simulink model "microduck_linear_state_feedback"  (R2026b)
settings: Solver=ode15s  StopTime=r.test.duration  MaxStep=r.p.cfg.sim.maxStep  RelTol=r.p.cfg.sim.relTol  AbsTol=r.p.cfg.sim.absTol
PreLoadFcn:
  | root=fileparts(get_param(bdroot,'FileName')); addpath(root,fullfile(root,'helpers')); md_expanded_cache;
PostLoadFcn:
  | md_sf_apply(bdroot);
InitFcn:
  | md_sf_apply(bdroot);
model workspace (MAT data in the model file):
  A = [0 0 0 0 0 0 0 0 0 0 0 0 ... (1296 elements, 36x36)]
  B = [0  0  0  0  0  0  0  0; 0  0  0  0  0  0  0  0; 0  0  0  0  0  0  0  0; 0  0  0  0  0  0  0  0; 0  0  0  0  0  0  0  0; 0  0  0  0  0  0  0  0; 0  0  0  0  0  0  0  0; 0  0  0  0  0  0  0  0; 0  0  0  0  0  0  0  0; 0  0  0  0  0  0  0  0; 0  0  0  0  0  0  0  0; 0  0  0  0  0  0  0  0; 0  0  0  0  0  0  0  0; 0  0  0  0  0  0  0  0; 0  0  0  0  0  0  0  0; 0  0  0  0  0  0  0  0; 0  0  0  0  0  0  0  0; 0  0  0  0  0  0  0  0; 0  0  0  0  0  0  0  0; 0  0  0  0  0  0  0  0; 0  0  0  0  0  0  0  0; 0  0  0  0  0  0  0  0; 0  0  0  0  0  0  0  0; 0  0  0  0  0  0  0  0; 0  0  0  0  0  0  0  0; 0  0  0  0  0  0  0  0; 0  0  0  0  0  0  0  0; 0  0  0  0  0  0  0  0; 18.3333333333  0  0  0  0  0  0  0; 0  18.3333333328  0  0  0  0  0  0; 0  0  18.3333333339  0  0  0  0  0; 0  0  0  18.3333333328  0  0  0  0; 0  0  0  0  18.3333333333  0  0  0; 0  0  0  0  0  18.3333333328  0  0; 0  0  0  0  0  0  18.3333333339  0; 0  0  0  0  0  0  0  18.3333333328]
  C = [0 0 0 0 0 0 0 0 0 0 0 0 ... (504 elements, 14x36)]
  E = [0  0  0  0  0  0; 0  0  0  0  0  0; 0  0  0  0  0  0; 0  0  0  0  0  0; 0  0  0  0  0  0; 0  0  0  0  0  0; 0  0  0  0  0  0; 0  0  0  0  0  0; 0  0  0  0  0  0; 0  0  0  0  0  0; 0  0  0  0  0  0; 0  0  0  0  0  0; 0  0  0  0  0  0; 0  0  0  0  0  0; 2.99982286451  -1.39842679811e-16  0.177414688657  -4.57651764544e-15  -30.0277204497  6.50739104523e-15; -1.58268629198e-16  2.89225820935  6.70083365122e-17  26.4522242149  3.51536253633e-15  -2.99721816856; 0.177414688663  8.37728579002e-17  1.49617665797  1.51751719319e-15  -1.96848927847  1.08542064426e-15; 6.08932332349e-15  -2.9843307487  6.98022045066e-16  -46.5047890403  -1.8610446411e-13  1033.95442638; -30.0277204497  3.01733642702e-15  -1.9684892784  9.66057478592e-14  670.762570803  -1.79597476519e-13; -2.99085236462e-15  26.4522273543  1.22764163289e-15  571.194337556  6.97130001697e-14  -46.7830781998; 4.28916538281e-15  -58.9426085695  -3.230112201e-15  -867.400266402  -9.48911648967e-14  29.6379320526; 93.8758569341  20.513888201  31.4835453095  429.750563248  -1381.35416373  -794.127195927; -48.639015031  -44.7564909477  -63.6327672593  -957.446876757  541.099997319  595.256445506; -27.6741686092  33.1017153167  46.5274762001  722.046276778  308.318673607  358.193155987; 4.44518421763e-15  -58.9426085695  -2.95924669915e-15  -867.400266402  -9.69858375627e-14  29.6379320526; 93.8758569341  -20.513888201  31.4835453095  -429.750563248  -1381.35416373  794.127195927; -48.639015031  44.7564909477  -63.6327672593  957.446876757  541.099997319  -595.256445506; -27.6741686092  -33.1017153167  46.5274762001  -722.046276778  308.318673607  -358.193155987; 0  0  0  0  0  0; 0  0  0  0  0  0; 0  0  0  0  0  0; 0  0  0  0  0  0; 0  0  0  0  0  0; 0  0  0  0  0  0; 0  0  0  0  0  0; 0  0  0  0  0  0]
  F_w = [0  0  0  0  0  0; 0  0  0  0  0  0; 0  0  0  0  0  0; 1.49835005027  0  0.0782612723698  0  3.51137069423  0; 2.66705636347e-18  1.56957414393  9.97031711871e-17  -2.1086255103  -9.94861602458e-17  -0.632877334553; 0.178876169343  0  1.49626291615  0  -1.98311843072  0; 0  0  0  0  0  0; 0  0  0  0  0  0; 0  0  0  0  0  0; 0  0  0  0  0  0; 0  0  0  0  0  0; 0  0  0  0  0  0; 0  0  0  0  0  0; 0  0  0  0  0  0]
  push_wrench = [1; 0; 0; 0; 0; 0]
  r.p.cfg.robot.gravity = [0; 0; -9.81]
  r.p.cfg.robot.hipHalfSpacing = 0.04
  r.p.cfg.robot.hipPitchDrop = 0.01
  r.p.cfg.robot.thighLength = 0.05
  r.p.cfg.robot.shinLength = 0.05
  r.p.cfg.robot.thighWidth = 0.025
  r.p.cfg.robot.shinWidth = 0.022
  r.p.cfg.robot.footLength = 0.054
  r.p.cfg.robot.footWidth = 0.041
  r.p.cfg.robot.footThickness = 0.012
  r.p.cfg.robot.soleDepth = 0.018
  r.p.cfg.robot.torsoDimensions = [0.09; 0.1; 0.14]
  r.p.cfg.robot.imuOffset = [0; 0; 0.05]
  r.p.cfg.robot.torsoCOM = [0; 0; 0.055]
  r.p.cfg.robot.carrierDimensions = [0.025; 0.025; 0.02]
  r.p.cfg.robot.massTorso = 0.5045154
  r.p.cfg.robot.massCarrier = 0.0287231
  r.p.cfg.robot.massThigh = 0.04315
  r.p.cfg.robot.massShin = 0.0215844
  r.p.cfg.robot.massFoot = 0.02646535
  r.p.cfg.robot.standingJointDeg = [0; -20; 40; -20; 0; -20; 40; -20]
  r.p.cfg.servo.kp = [0.55; 0.55; 0.55; 0.55; 0.55; 0.55; 0.55; 0.55]
  r.p.cfg.servo.kd = [0; 0; 0; 0; 0; 0; 0; 0]
  r.p.cfg.servo.timeConstant = [0.03; 0.03; 0.03; 0.03; 0.03; 0.03; 0.03; 0.03]
  r.p.cfg.servo.maxTorque = [0.6; 0.6; 0.6; 0.6; 0.6; 0.6; 0.6; 0.6]
  r.p.cfg.servo.jointDamping = [0.053; 0.053; 0.053; 0.053; 0.053; 0.053; 0.053; 0.053]
  r.p.cfg.servo.minCommandDeg = [-20.0535228296; -57.2957795131; 2.86478897565; -45.8366236105; -20.0535228296; -57.2957795131; 2.86478897565; -45.8366236105]
  r.p.cfg.servo.maxCommandDeg = [20.0535228296; 34.3774677078; 85.9436692696; 45.8366236105; 20.0535228296; 34.3774677078; 85.9436692696; 45.8366236105]
  r.p.cfg.contact.stiffness = 4000
  r.p.cfg.contact.damping = 12
  r.p.cfg.contact.friction = 0.6
  r.p.cfg.contact.frictionVelocity = 0.005
  r.p.cfg.sim.sampleTime = 0.02
  r.p.cfg.sim.stopTime = 3
  r.p.cfg.sim.maxStep = 0.002
  r.p.cfg.sim.relTol = 1e-06
  r.p.cfg.sim.absTol = 1e-08
  r.p.cfg.stop.enabled = 1
  r.p.cfg.stop.maxTiltDeg = 20
  r.p.cfg.stop.minHipHeight = 0.06
  r.p.cfg.measurements.includeJointVelocity = 0
  r.p.g = [0; 0; -9.81]
  r.p.nq = 14
  r.p.S = [0  0  0  0  0  0  0  0; 0  0  0  0  0  0  0  0; 0  0  0  0  0  0  0  0; 0  0  0  0  0  0  0  0; 0  0  0  0  0  0  0  0; 0  0  0  0  0  0  0  0; 1  0  0  0  0  0  0  0; 0  1  0  0  0  0  0  0; 0  0  1  0  0  0  0  0; 0  0  0  1  0  0  0  0; 0  0  0  0  1  0  0  0; 0  0  0  0  0  1  0  0; 0  0  0  0  0  0  1  0; 0  0  0  0  0  0  0  1]
  r.p.kp = [0.55; 0.55; 0.55; 0.55; 0.55; 0.55; 0.55; 0.55]
  r.p.kd = [0; 0; 0; 0; 0; 0; 0; 0]
  r.p.Ta = [0.03; 0.03; 0.03; 0.03; 0.03; 0.03; 0.03; 0.03]
  r.p.tauMax = [0.6; 0.6; 0.6; 0.6; 0.6; 0.6; 0.6; 0.6]
  r.p.bjoint = [0.053; 0.053; 0.053; 0.053; 0.053; 0.053; 0.053; 0.053]
  r.p.jointMin = [-0.35; -1; 0.05; -0.8; -0.35; -1; 0.05; -0.8]
  r.p.jointMax = [0.35; 0.6; 1.5; 0.8; 0.35; 0.6; 1.5; 0.8]
  r.p.kn = 4000
  r.p.cn = 12
  r.p.mu = 0.6
  r.p.vs = 0.005
  r.p.imuOffset = [0; 0; 0.05]
  r.p.parent = [0 1 2 3 4 1 6 7 8]
  r.p.jointIndex = [0 7 8 9 10 11 12 13 14]
  r.p.axis = [0  1  0  0  0  1  0  0  0; 0  0  1  1  1  0  1  1  1; 0  0  0  0  0  0  0  0  0]
  r.p.offset = [0  0  0  0  0  0  0  0  0; 0  0.04  0  0  0  -0.04  0  0  0; 0  0  -0.01  -0.05  -0.05  0  -0.01  -0.05  -0.05]
  r.p.mass = [0.5045154 0.0287231 0.04315 0.0215844 0.02646535 0.0287231 0.04315 0.0215844 0.02646535]
  r.p.com = [0  0  0  0  0  0  0  0  0; 0  0  0  0  0  0  0  0  0; 0.055  -0.005  -0.025  -0.025  -0.012  -0.005  -0.025  -0.025  -0.012]
  r.p.inertia = reshape([0.00124447132 0 0 0 0.001164589715 0 0 0 0.000760977395 2.45343145833e-06 0 0 0 2.45343145833e-06 0 0 0 2.99198958333e-06 1.12369791667e-05 0 0 0 1.12369791667e-05 0 0 0 4.49479166667e-06 5.3673208e-06 0 0 0 5.3673208e-06 0 0 0 1.7411416e-06 4.02493864583e-06 0 0 0 6.74866425e-06 0 0 0 1.01384344958e-05 2.45343145833e-06 0 0 0 2.45343145833e-06 0 0 0 2.99198958333e-06 1.12369791667e-05 0 0 0 1.12369791667e-05 0 0 0 4.49479166667e-06 5.3673208e-06 0 0 0 5.3673208e-06 0 0 0 1.7411416e-06 4.02493864583e-06 0 0 0 6.74866425e-06 0 0 0 1.01384344958e-05], [3 3 9])
  r.p.footBodies = [5 9]
  r.p.corners = [-0.027  -0.027  0.027  0.027; -0.0205  0.0205  -0.0205  0.0205; -0.018  -0.018  -0.018  -0.018]
  r.p.qnom = [0; 0; 0.121741068879; 0; 0; 0; 0; -0.349065850399; 0.698131700798; -0.349065850399; 0; -0.349065850399; 0.698131700798; -0.349065850399]
  r.p.trimResidual = 3.34843264227e-13
  r.p.trimNormal = [0.86015562883; 0.86015562883; 0.96538996892; 0.96538996892; 0.86015562883; 0.86015562883; 0.96538996892; 0.96538996892]
  r.p.xeq = [0; 0; 0.121741054404; 0; 0.00048719603821; 6.28632250353e-17; 0; -0.349065850399; 0.698131700798; -0.349065850399; 0; -0.349065850399; 0.698131700798; -0.349065850399; 0; 0; 0; 0; 0; 0; 0; 0; 0; 0; 0; 0; 0; 0; 5.52116353176e-16; 7.90529085794e-05; -0.0506100270862; 0.00565215320243; 5.52116353176e-16; 7.90529085794e-05; -0.0506100270862; 0.00565215320243]
  r.p.ueq = [1.00384791487e-15; -0.348922117838; 0.606113469732; -0.338789208213; 1.00384791487e-15; -0.348922117838; 0.606113469732; -0.338789208213]
  r.lin.A = [0 0 0 0 0 0 0 0 0 0 0 0 ... (1296 elements, 36x36)]
  r.lin.B = [0  0  0  0  0  0  0  0; 0  0  0  0  0  0  0  0; 0  0  0  0  0  0  0  0; 0  0  0  0  0  0  0  0; 0  0  0  0  0  0  0  0; 0  0  0  0  0  0  0  0; 0  0  0  0  0  0  0  0; 0  0  0  0  0  0  0  0; 0  0  0  0  0  0  0  0; 0  0  0  0  0  0  0  0; 0  0  0  0  0  0  0  0; 0  0  0  0  0  0  0  0; 0  0  0  0  0  0  0  0; 0  0  0  0  0  0  0  0; 0  0  0  0  0  0  0  0; 0  0  0  0  0  0  0  0; 0  0  0  0  0  0  0  0; 0  0  0  0  0  0  0  0; 0  0  0  0  0  0  0  0; 0  0  0  0  0  0  0  0; 0  0  0  0  0  0  0  0; 0  0  0  0  0  0  0  0; 0  0  0  0  0  0  0  0; 0  0  0  0  0  0  0  0; 0  0  0  0  0  0  0  0; 0  0  0  0  0  0  0  0; 0  0  0  0  0  0  0  0; 0  0  0  0  0  0  0  0; 18.3333333333  0  0  0  0  0  0  0; 0  18.3333333328  0  0  0  0  0  0; 0  0  18.3333333339  0  0  0  0  0; 0  0  0  18.3333333328  0  0  0  0; 0  0  0  0  18.3333333333  0  0  0; 0  0  0  0  0  18.3333333328  0  0; 0  0  0  0  0  0  18.3333333339  0; 0  0  0  0  0  0  0  18.3333333328]
  r.lin.C = [0  0  0  0  0  0  0  0  0  0  0  0  0  0  0  0  0  -0.000487196018936  0  1  0  0  0  0  0  0  0  0  0  0  0  0  0  0  0  0; 0  0  0  0  0  0  0  0  0  0  0  0  0  0  0  0  0  6.28632175747e-17  1  5.73971850987e-36  0  0  0  0  0  0  0  0  0  0  0  0  0  0  0  0; 0  0  0  0  0  0  0  0  0  0  0  0  0  0  0  0  0  0.99999988132  -6.28632250353e-17  0  0  0  0  0  0  0  0  0  0  0  0  0  0  0  0  0; 0  0  9265.46457746  0  130.165054704  -6.84001466578e-08  -2.07256087292e-09  69.3951978499  144.565706863  64.1932730965  -2.10595429984e-09  69.3951978499  144.565706863  64.1932730965  74.0137947271  0  27.7963937321  6.20163642662e-11  -8.63881750136  -1.78676518026e-10  2.86229373536e-10  -5.26342586956  -0.830679547445  0.178354369236  2.57172755314e-10  -5.26342586956  -0.830679547439  0.178354369236  0  24.7927989485  -21.5530077617  -12.2808996456  0  24.7927989485  -21.5530077617  -12.2808996456; 0  0  -7.82627372827e-11  -1.15367357622e-10  1.01085418767e-08  272.89136386  112.119374165  10.1316970194  18.6847145316  9.9177480342  112.119374165  -10.1316970296  -18.6847145316  -9.9177480442  8.21255251386e-14  515.113047543  -3.2086916701e-11  0.947725865768  -3.57478340115e-11  63.6596220389  32.5958842775  -0.557372026813  -0.482069576678  0.0855967928727  32.5958842776  0.55737202677  0.482069576771  -0.0855967928114  -15.5718784225  -0.992982191643  3.13034753722  -2.99186872359  -15.5718784225  0.992982191643  -3.13034753722  2.99186872359; 0  0  -13045.3812466  0  -291.511055468  1.00364161426e-07  4.4408920985e-09  -145.399577004  -260.915887701  -143.957256833  4.4408920985e-09  -145.399577003  -260.915887701  -143.957256832  -165.916252803  0  -39.1361437391  8.881784197e-10  19.3664195969  0  8.881784197e-10  7.18267224187  7.99488262881  -1.40613470379  0  7.18267224276  7.99488262881  -1.40613470467  0  31.5292775177  -63.6564564429  46.5139879342  0  31.5292775177  -63.6564564429  46.5139879342]
  r.lin.D = [0  0  0  0  0  0  0  0; 0  0  0  0  0  0  0  0; 0  0  0  0  0  0  0  0; 0  0  0  0  0  0  0  0; 0  0  0  0  0  0  0  0; 0  0  0  0  0  0  0  0]
  r.lin.C_with_joint_angles = [0 0 0 0 0 0 0 0 0 0 0 0 ... (504 elements, 14x36)]
  r.lin.D_with_joint_angles = [0  0  0  0  0  0  0  0; 0  0  0  0  0  0  0  0; 0  0  0  0  0  0  0  0; 0  0  0  0  0  0  0  0; 0  0  0  0  0  0  0  0; 0  0  0  0  0  0  0  0; 0  0  0  0  0  0  0  0; 0  0  0  0  0  0  0  0; 0  0  0  0  0  0  0  0; 0  0  0  0  0  0  0  0; 0  0  0  0  0  0  0  0; 0  0  0  0  0  0  0  0; 0  0  0  0  0  0  0  0; 0  0  0  0  0  0  0  0]
  r.lin.C_measurements = [0 0 0 0 0 0 0 0 0 0 0 0 ... (504 elements, 14x36)]
  r.lin.D_measurements = [0  0  0  0  0  0  0  0; 0  0  0  0  0  0  0  0; 0  0  0  0  0  0  0  0; 0  0  0  0  0  0  0  0; 0  0  0  0  0  0  0  0; 0  0  0  0  0  0  0  0; 0  0  0  0  0  0  0  0; 0  0  0  0  0  0  0  0; 0  0  0  0  0  0  0  0; 0  0  0  0  0  0  0  0; 0  0  0  0  0  0  0  0; 0  0  0  0  0  0  0  0; 0  0  0  0  0  0  0  0; 0  0  0  0  0  0  0  0]
  r.lin.xeq = [0; 0; 0.121741054404; 0; 0.00048719603821; 6.28632250353e-17; 0; -0.349065850399; 0.698131700798; -0.349065850399; 0; -0.349065850399; 0.698131700798; -0.349065850399; 0; 0; 0; 0; 0; 0; 0; 0; 0; 0; 0; 0; 0; 0; 5.52116353176e-16; 7.90529085794e-05; -0.0506100270862; 0.00565215320243; 5.52116353176e-16; 7.90529085794e-05; -0.0506100270862; 0.00565215320243]
  r.lin.ueq = [1.00384791487e-15; -0.348922117838; 0.606113469732; -0.338789208213; 1.00384791487e-15; -0.348922117838; 0.606113469732; -0.338789208213]
  r.lin.yeq = [0; 0; 0; -0.00477939294573; 2.9613909167e-15; 9.80999883575]
  r.lin.yeq_measurements = [0; 0; 0; -0.00477939294573; 2.9613909167e-15; 9.80999883575; 0; -0.349065850399; 0.698131700798; -0.349065850399; 0; -0.349065850399; 0.698131700798; -0.349065850399]
  r.lin.stateScale = [0.01; 0.01; 0.01; 0.1; 0.1; 0.1; 0.1; 0.1; 0.1; 0.1; 0.1; 0.1; 0.1; 0.1; 0.1; 0.1; 0.1; 1; 1; 1; 1; 1; 1; 1; 1; 1; 1; 1; 0.1; 0.1; 0.1; 0.1; 0.1; 0.1; 0.1; 0.1]
  r.lin.controlSampleTime = 0.02
  r.aux.E = [0  0  0  0  0  0; 0  0  0  0  0  0; 0  0  0  0  0  0; 0  0  0  0  0  0; 0  0  0  0  0  0; 0  0  0  0  0  0; 0  0  0  0  0  0; 0  0  0  0  0  0; 0  0  0  0  0  0; 0  0  0  0  0  0; 0  0  0  0  0  0; 0  0  0  0  0  0; 0  0  0  0  0  0; 0  0  0  0  0  0; 2.99982286451  -1.39842679811e-16  0.177414688657  -4.57651764544e-15  -30.0277204497  6.50739104523e-15; -1.58268629198e-16  2.89225820935  6.70083365122e-17  26.4522242149  3.51536253633e-15  -2.99721816856; 0.177414688663  8.37728579002e-17  1.49617665797  1.51751719319e-15  -1.96848927847  1.08542064426e-15; 6.08932332349e-15  -2.9843307487  6.98022045066e-16  -46.5047890403  -1.8610446411e-13  1033.95442638; -30.0277204497  3.01733642702e-15  -1.9684892784  9.66057478592e-14  670.762570803  -1.79597476519e-13; -2.99085236462e-15  26.4522273543  1.22764163289e-15  571.194337556  6.97130001697e-14  -46.7830781998; 4.28916538281e-15  -58.9426085695  -3.230112201e-15  -867.400266402  -9.48911648967e-14  29.6379320526; 93.8758569341  20.513888201  31.4835453095  429.750563248  -1381.35416373  -794.127195927; -48.639015031  -44.7564909477  -63.6327672593  -957.446876757  541.099997319  595.256445506; -27.6741686092  33.1017153167  46.5274762001  722.046276778  308.318673607  358.193155987; 4.44518421763e-15  -58.9426085695  -2.95924669915e-15  -867.400266402  -9.69858375627e-14  29.6379320526; 93.8758569341  -20.513888201  31.4835453095  -429.750563248  -1381.35416373  794.127195927; -48.639015031  44.7564909477  -63.6327672593  957.446876757  541.099997319  -595.256445506; -27.6741686092  -33.1017153167  46.5274762001  -722.046276778  308.318673607  -358.193155987; 0  0  0  0  0  0; 0  0  0  0  0  0; 0  0  0  0  0  0; 0  0  0  0  0  0; 0  0  0  0  0  0; 0  0  0  0  0  0; 0  0  0  0  0  0; 0  0  0  0  0  0]
  r.aux.Fw = [0  0  0  0  0  0; 0  0  0  0  0  0; 0  0  0  0  0  0; 1.49835005027  0  0.0782612723698  0  3.51137069423  0; 2.66705636347e-18  1.56957414393  9.97031711871e-17  -2.1086255103  -9.94861602458e-17  -0.632877334553; 0.178876169343  0  1.49626291615  0  -1.98311843072  0; 0  0  0  0  0  0; 0  0  0  0  0  0; 0  0  0  0  0  0; 0  0  0  0  0  0; 0  0  0  0  0  0; 0  0  0  0  0  0; 0  0  0  0  0  0; 0  0  0  0  0  0]
  r.feedback.K = [8.70410247674e-16 -0.000482616394029 -0.000818546928294 -0.00100799621853 -3.20893583014e-15 -0.000482616394022 -0.000818546928299 -0.00100799621853 3.94214592664e-14 -0.0216180096191 -0.0366654667942 -0.0451515369514 ... (264 elements, 8x33)]
  r.feedback.poles = [-0.173706973501+0.0790896944051i; -0.173706973501-0.0790896944051i; -0.014115987547+0.0894236107172i; -0.014115987547-0.0894236107172i; 0.672250176228+0.561912229918i; 0.672250176228-0.561912229918i; -0.0822703613827+0.0594677475137i; -0.0822703613827-0.0594677475137i; 0.0992828819218+0i; 0.891684694096+0i; 0.886920436717+0i; 0.735487634412+0.114439990771i; 0.735487634412-0.114439990771i; 0.717373000186+0.112026826557i; 0.717373000186-0.112026826557i; 0.976285709758+0i; 0.980198673307+0i; 0.721801481118+0.118511971968i; 0.721801481118-0.118511971968i; 0.482156928981+0i; 0.480371127775+0i; 0.492850316995+0i; 0.515715029329+0i; 0.514305187301+0i; 2.94698823164e-09+0i; -5.41379190099e-16+0i; 1.47117542566e-16+0i; 1.11020150478e-17+9.9609496806e-17i; 1.11020150478e-17-9.9609496806e-17i; -2.28360718307e-17+3.66102795761e-17i; -2.28360718307e-17-3.66102795761e-17i; 2.99664398283e-17+2.17653008708e-17i; 2.99664398283e-17-2.17653008708e-17i]
  r.feedback.requestedPoles = [-0.173706973501+0.0790896944051i; -0.173706973501-0.0790896944051i; -0.014115987547+0.0894236107172i; -0.014115987547-0.0894236107172i; 0.672250176228+0.561912229918i; 0.672250176228-0.561912229918i; -0.0822703613827+0.0594677475137i; -0.0822703613827-0.0594677475137i; 0.0992828819218+0i; 0.891684694096+0i; 0.735487634412+0.114439990771i; 0.735487634412-0.114439990771i; 0.717373000186+0.112026826557i; 0.717373000186-0.112026826557i; 0.721801481118+0.118511971968i; 0.721801481118-0.118511971968i; 0.482156928981+0i; 0.480371127775+0i; 0.492850316995+0i; 0.515715029329+0i; 0.514305187301+0i; 2.9469884e-09+0i; 5.84077967475e-15+0i; -2.65521112042e-15+2.05477564382e-15i; -2.65521112042e-15-2.05477564382e-15i; 3.09349036794e-15+0i; 9.13638941562e-16+0i; -4.87155219894e-16+0i; 1.66967134563e-16+2.25567004766e-16i; 1.66967134563e-16-2.25567004766e-16i; 0.886920436717+0i; 0.976285709758+0i; 0.980198673307+0i]
  r.feedback.assignedSlowPoles = [0.886920436717; 0.976285709758; 0.980198673307]
  r.feedback.retainedFastPoleCount = 30
  r.feedback.poleMatchError = 1.58095758707e-13
  r.feedback.placementPrecision = 15
  r.feedback.radius = 0.980198673307
  r.feedback.reference = [0; 0]
  r.feedback.maxCorrectionRad = 0.13962634016
  r.feedback.sampleTime = 0.02
  r.observer.Ad = [-0.226035158295 0.0607901151539 1.20046417563e-11 -1.4732593899e-11 -0.156351729745 0.138229107162 0.0857639497085 -1.47317675914e-11 -0.156351729733 0.138229107138 0.0857639497232 1.19581922834 ... (1089 elements, 33x33)]
  r.observer.Bd = [-1.57872286761e-12 -2.75043555489e-12 -0.0544924598499 0.0922096305921 -0.0255771207666 0.0488604655049 -0.0163542439887 0.087766164084 0.0255771207875 -0.0488604655276 0.016354243994 1.82708257098e-11 ... (264 elements, 33x8)]
  r.observer.C = [0 0 0 9.44491801984 -7.97785293402e-14 -13.2980440841 0 0 0 0 0 0 ... (462 elements, 14x33)]
  r.observer.D = [0  0  0  0  0  0  0  0; 0  0  0  0  0  0  0  0; 0  0  0  0  0  0  0  0; 0  0  0  0  0  0  0  0; 0  0  0  0  0  0  0  0; 0  0  0  0  0  0  0  0; 0  0  0  0  0  0  0  0; 0  0  0  0  0  0  0  0; 0  0  0  0  0  0  0  0; 0  0  0  0  0  0  0  0; 0  0  0  0  0  0  0  0; 0  0  0  0  0  0  0  0; 0  0  0  0  0  0  0  0; 0  0  0  0  0  0  0  0]
  r.observer.L = [-7.01418682646e-12 8.04628712517e-11 0.0643927661333 0.24278751739 0.0372639622641 -0.0756135571544 0.0275453071133 0.242787517394 -0.0372639605356 0.07561355728 -0.0275453090267 5.98286207219e-10 ... (462 elements, 33x14)]
  r.observer.errorMatrix = [-0.251020245761 0.799832731146 2.38563787379e-09 7.04126391556e-09 2.62313977309 0.267993545053 -3.41200716347 7.0849640839e-09 2.62313976989 0.267993551207 -3.41200716574 3.40012488569 ... (1089 elements, 33x33)]
  r.observer.poles = [-0.173706973501+0.0790896944051i; -0.173706973501-0.0790896944051i; -0.014115987547+0.0894236107172i; -0.014115987547-0.0894236107172i; -0.0822703613827+0.0594677475137i; -0.0822703613827-0.0594677475137i; 0.0992828819218+0i; 0.717373000186+0.112026826557i; 0.717373000186-0.112026826557i; 0.721801481118+0.118511971968i; 0.721801481118-0.118511971968i; 0.670320046036+0i; 0.482156928981+0i; 0.582748252374+0i; 0.59452054797+0i; 0.631283645507+0i; 0.657046819815+0i; 0.644036421083+0i; 0.618783391806+0i; 0.606530659713+0i; 0.480371127775+0i; 0.492850316995+0i; 0.514305187301+0i; 0.515715029329+0i; 2.94698765516e-09+0i; 1.91663560711e-14+0i; -6.86720396472e-15+0i; -3.48279432533e-16+9.37889198838e-16i; -3.48279432533e-16-9.37889198838e-16i; 7.85859192971e-16+3.70757158126e-16i; 7.85859192971e-16-3.70757158126e-16i; -2.4574281643e-16+0i; 2.80192628595e-16+0i]
  r.observer.continuousA = [0 0 0 0 0 0 0 0 0 0 0 2088.98331426 ... (1089 elements, 33x33)]
  r.observer.continuousB = [0  0  0  0  0  0  0  0; 0  0  0  0  0  0  0  0; 0  0  0  0  0  0  0  0; 0  0  0  0  0  0  0  0; 0  0  0  0  0  0  0  0; 0  0  0  0  0  0  0  0; 0  0  0  0  0  0  0  0; 0  0  0  0  0  0  0  0; 0  0  0  0  0  0  0  0; 0  0  0  0  0  0  0  0; 0  0  0  0  0  0  0  0; 0  0  0  0  0  0  0  0; 0  0  0  0  0  0  0  0; 0  0  0  0  0  0  0  0; 0  0  0  0  0  0  0  0; 0  0  0  0  0  0  0  0; 0  0  0  0  0  0  0  0; 0  0  0  0  0  0  0  0; 0  0  0  0  0  0  0  0; 0  0  0  0  0  0  0  0; 0  0  0  0  0  0  0  0; 0  0  0  0  0  0  0  0; 0  0  0  0  0  0  0  0; 0  0  0  0  0  0  0  0; 0  0  0  0  0  0  0  0; 183.333333333  0  0  0  0  0  0  0; 0  183.333333328  0  0  0  0  0  0; 0  0  183.333333339  0  0  0  0  0; 0  0  0  183.333333328  0  0  0  0; 0  0  0  0  183.333333333  0  0  0; 0  0  0  0  0  183.333333328  0  0; 0  0  0  0  0  0  183.333333339  0; 0  0  0  0  0  0  0  183.333333328]
  r.observer.y0 = [0; 0; 0; -0.00477939294573; 2.9613909167e-15; 9.80999883575; 0; -0.349065850399; 0.698131700798; -0.349065850399; 0; -0.349065850399; 0.698131700798; -0.349065850399]
  r.observer.yScale = [1; 1; 1; 9.81; 9.81; 9.81; 0.1; 0.1; 0.1; 0.1; 0.1; 0.1; 0.1; 0.1]
  r.observer.keep = [3 5 6 7 8 9 10 11 12 13 14 15 16 17 18 19 20 21 22 23 24 25 26 27 28 29 30 31 32 33 34 35 36]
  r.observer.S = [0.01 0 0 0 0 0 0 0 0 0 0 0 ... (1089 elements, 33x33)]
  r.observer.settings.initialAngleErrorDeg = [0.5; 1]
  r.observer.settings.slowModeCutoffRate = 15
  r.observer.settings.firstDecayRate = 20
  r.observer.settings.decayRateSpacing = 1
  r.observer.settings.initialEstimateDelta = [0; 0; 0; 0; 0.0174532925199; 0.00872664625997; 0; 0; 0; 0; 0; 0; 0; 0; 0; 0; 0; 0; 0; 0; 0; 0; 0; 0; 0; 0; 0; 0; 0; 0; 0; 0; 0; 0; 0; 0]
  r.observer.sampleTime = 0.02
  r.observer.requestedSlowPoles = [0.670320046036 0.657046819815 0.644036421083 0.631283645507 0.618783391806 0.606530659713 0.59452054797 0.582748252374]
  r.observer.retainedFastPoleCount = 25
  r.observer.placementPrecision = 14
  r.test.duration = 3
  r.test.pushForce = [1; 0; 0]
  r.test.pushMoment = [0; 0; 0]
  r.test.pushCentre = 0.2
  r.test.pushWidth = 0.02
  r.test.pushEnabled = 1
  r.test.pushPointBody = [0; 0; 0]
  r.H = [0  0  1  0  0  0  0  0  0  0  0  0  0  0  0  0  0  0  0  0  0  0  0  0  0  0  0  0  0  0  0  0  0; 0  1  0  0  0  0  0  0  0  0  0  0  0  0  0  0  0  0  0  0  0  0  0  0  0  0  0  0  0  0  0  0  0]
  r.sharedConfiguration.test.duration = 3
  r.sharedConfiguration.test.pushForce = [1; 0; 0]
  r.sharedConfiguration.test.pushMoment = [0; 0; 0]
  r.sharedConfiguration.test.pushCentre = 0.2
  r.sharedConfiguration.test.pushWidth = 0.02
  r.sharedConfiguration.sampleTime = 0.02
  r.sharedConfiguration.observer.initialAngleErrorDeg = [0.5; 1]
  r.sharedConfiguration.observer.slowModeCutoffRate = 15
  r.sharedConfiguration.observer.firstDecayRate = 20
  r.sharedConfiguration.observer.decayRateSpacing = 1
  r.sharedConfiguration.robot.gravity = [0; 0; -9.81]
  r.sharedConfiguration.robot.hipHalfSpacing = 0.04
  r.sharedConfiguration.robot.hipPitchDrop = 0.01
  r.sharedConfiguration.robot.thighLength = 0.05
  r.sharedConfiguration.robot.shinLength = 0.05
  r.sharedConfiguration.robot.thighWidth = 0.025
  r.sharedConfiguration.robot.shinWidth = 0.022
  r.sharedConfiguration.robot.footLength = 0.054
  r.sharedConfiguration.robot.footWidth = 0.041
  r.sharedConfiguration.robot.footThickness = 0.012
  r.sharedConfiguration.robot.soleDepth = 0.018
  r.sharedConfiguration.robot.torsoDimensions = [0.09; 0.1; 0.14]
  r.sharedConfiguration.robot.imuOffset = [0; 0; 0.05]
  r.sharedConfiguration.robot.torsoCOM = [0; 0; 0.055]
  r.sharedConfiguration.robot.carrierDimensions = [0.025; 0.025; 0.02]
  r.sharedConfiguration.robot.massTorso = 0.5045154
  r.sharedConfiguration.robot.massCarrier = 0.0287231
  r.sharedConfiguration.robot.massThigh = 0.04315
  r.sharedConfiguration.robot.massShin = 0.0215844
  r.sharedConfiguration.robot.massFoot = 0.02646535
  r.sharedConfiguration.robot.standingJointDeg = [0; -20; 40; -20; 0; -20; 40; -20]
  r.sharedConfiguration.servo.kp = [0.55; 0.55; 0.55; 0.55; 0.55; 0.55; 0.55; 0.55]
  r.sharedConfiguration.servo.kd = [0; 0; 0; 0; 0; 0; 0; 0]
  r.sharedConfiguration.servo.timeConstant = [0.03; 0.03; 0.03; 0.03; 0.03; 0.03; 0.03; 0.03]
  r.sharedConfiguration.servo.maxTorque = [0.6; 0.6; 0.6; 0.6; 0.6; 0.6; 0.6; 0.6]
  r.sharedConfiguration.servo.jointDamping = [0.053; 0.053; 0.053; 0.053; 0.053; 0.053; 0.053; 0.053]
  r.sharedConfiguration.servo.minCommandDeg = [-20.0535228296; -57.2957795131; 2.86478897565; -45.8366236105; -20.0535228296; -57.2957795131; 2.86478897565; -45.8366236105]
  r.sharedConfiguration.servo.maxCommandDeg = [20.0535228296; 34.3774677078; 85.9436692696; 45.8366236105; 20.0535228296; 34.3774677078; 85.9436692696; 45.8366236105]
  r.sharedConfiguration.contact.stiffness = 4000
  r.sharedConfiguration.contact.damping = 12
  r.sharedConfiguration.contact.friction = 0.6
  r.sharedConfiguration.contact.frictionVelocity = 0.005
  r.sharedConfiguration.feedback.assignedDecayRates = [6; 1; 1.2]
  r.sharedConfiguration.feedback.slowModeCutoffRate = 2.5
  r.sharedConfiguration.feedback.poleMatchTolerance = 1e-06
  r.sharedConfiguration.feedback.maxCorrectionDeg = 8
  r.sharedConfiguration.solver.maxStep = 0.002
  r.sharedConfiguration.solver.relTol = 1e-06
  r.sharedConfiguration.solver.absTol = 1e-08
  r.sharedConfiguration.validity.maxTiltDeg = 20
  r.sharedConfiguration.validity.minHipHeight = 0.06
  r.sharedVersion = 1
  r.mode = 'linear'
  u_eq = [1.00384791487e-15; -0.348922117838; 0.606113469732; -0.338789208213; 1.00384791487e-15; -0.348922117838; 0.606113469732; -0.338789208213]
  x_eq = [0; 0; 0.121741054404; 0; 0.00048719603821; 6.28632250353e-17; 0; -0.349065850399; 0.698131700798; -0.349065850399; 0; -0.349065850399; 0.698131700798; -0.349065850399; 0; 0; 0; 0; 0; 0; 0; 0; 0; 0; 0; 0; 0; 0; 5.52116353176e-16; 7.90529085794e-05; -0.0506100270862; 0.00565215320243; 5.52116353176e-16; 7.90529085794e-05; -0.0506100270862; 0.00565215320243]
  y_eq = [0; 0; 0; -0.00477939294573; 2.9613909167e-15; 9.80999883575; 0; -0.349065850399; 0.698131700798; -0.349065850399; 0; -0.349065850399; 0.698131700798; -0.349065850399]
settings Model: Creator=parve  LastModifiedBy=parve

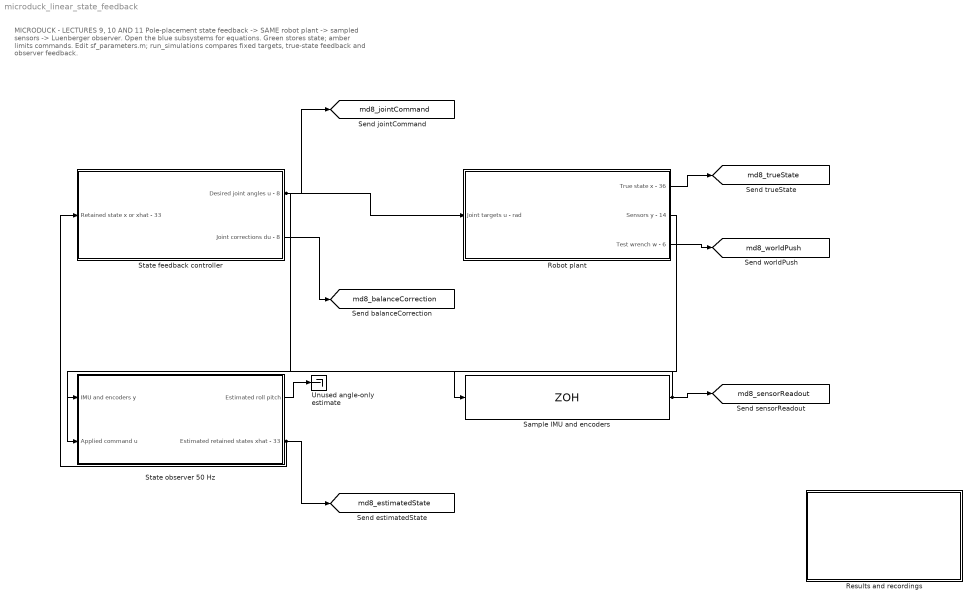
== system microduck_linear_state_feedback ==
  note: MICRODUCK - LECTURES 9, 10 AND 11
      | Pole-placement state feedback -> SAME robot plant -> sampled sensors -> Luenberger observer.
      | Open the blue subsystems for equations. Green stores state; amber limits commands.
      | Edit sf_parameters.m; run_simulations compares fixed targets, true-state feedback and observer feedback.
  Results and recordings : Subsystem  Description=|
      | RESULTS AND RECORDINGS
      | 
      | Purpose: record signals for plotting and comparison. These blocks do not control the robot.
      | trueState: actual motion; estimatedState: observer output; jointCommand: applied targets.
      | sensorReadout, worldPush and balanceCorrection complete the experiment records.
      mask help:
      | RESULTS AND RECORDINGS
      |
      | Purpose: record signals for plotting and comparison. These blocks do not control the robot.
      | trueState: actual motion; estimatedState: observer output; jointCommand: applied targets.
      | sensorReadout, worldPush and balanceCorrection complete the experiment records.
      settings: OpenFcn=open_system(gcb,'force');
      mask Display: disp('Results and recordings');
  Robot plant : Subsystem  Description=|
      | LINEAR PLANT - SMALL CHANGES ABOUT STANDING
      | 
      | Purpose: approximate the robot near its standing equilibrium.
      | State derivative = A * state deviation + B * command deviation + E * push.
      | The integrator stores state deviations; add standing offsets to reconstruct physical outputs.
      mask help:
      | LINEAR PLANT - SMALL CHANGES ABOUT STANDING
      |
      | Purpose: approximate the robot near its standing equilibrium.
      | State derivative = A * state deviation + B * command deviation + E * push.
      | The integrator stores state deviations; add standing offsets to reconstruct physical outputs.
      settings: OpenFcn=open_system(gcb,'force');
      mask Display: disp('Robot plant');
  Sample IMU and encoders : ZeroOrderHold  Description=|  SampleTime=r.observer.sampleTime
      | Sample IMU and encoders
      | 
      | WHAT THIS BLOCK DOES
      | Samples the sensor signal every 0.02 s and holds that measurement between samples, representing the 50 Hz readout clock.
      | 
      | FOLDER CONTEXT
      | MICRODUCK BALANCE - START HERE
      | 
      | Follow the loop: state-feedback controller -> robot plant -> sampled sensors -> observer -> PID.
      | Open a folder for its purpose, signal meanings and equations. Green blocks store state; amber blocks limit signals.
      | The controller and observer update at 50 Hz. Results are recorded separately on the right.
  State feedback controller : Subsystem  Description=Lecture 9 pole-placement feedback. Normalize standing state deviations, apply -K, limit offsets, and add standing joint targets.
      settings: OpenFcn=open_system(gcb,'force');
      mask Display: disp('State feedback controller\nLecture 9: pole placement')
  State observer 50 Hz : Subsystem  Description=|
      | Lecture 10 Luenberger observer, sampled as in Lecture 11.
      | zhat[k+1]=Ad zhat[k]+Bd du[k]+L(yn[k]-Cn zhat[k]).
      | The same applied joint target is sent to both plant and observer.
      settings: OpenFcn=open_system(gcb,'force');
      mask Display: disp('State observer\nLuenberger pole placement')
  Unused angle-only estimate : Terminator
  tag scope: md8_balanceCorrection=global, md8_estimatedState=global, md8_jointCommand=global, md8_sensorReadout=global, md8_trueState=global, md8_worldPush=global
  wires:
  State feedback controller/1(Desired joint angles u - 8) -> Robot plant/1(Joint targets u - rad), State observer 50 Hz/2(Applied command u), [md8_jointCommand]
  State feedback controller/2(Joint corrections du - 8) -> [md8_balanceCorrection]
  Robot plant/1(True state x - 36) -> [md8_trueState]
  Robot plant/2(Sensors y - 14) -> Sample IMU and encoders/1
  Robot plant/3(Test wrench w - 6) -> [md8_worldPush]
  Sample IMU and encoders/1 -> State observer 50 Hz/1(IMU and encoders y), [md8_sensorReadout]
  State observer 50 Hz/2(Estimated retained states xhat - 33) -> State feedback controller/1(Retained state x or xhat - 33), [md8_estimatedState]
  State observer 50 Hz/1(Estimated roll pitch) -> Unused angle-only estimate/1

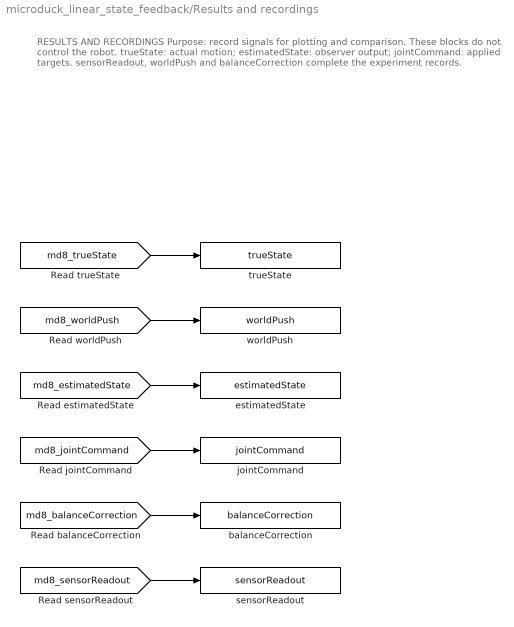
== system microduck_linear_state_feedback/Results and recordings ==
  note: RESULTS AND RECORDINGS
      |
      | Purpose: record signals for plotting and comparison. These blocks do not control the robot.
      | trueState: actual motion; estimatedState: observer output; jointCommand: applied targets.
      | sensorReadout, worldPush and balanceCorrection complete the experiment records.
  balanceCorrection : ToWorkspace  VariableName=balanceCorrection  SaveFormat=Timeseries  SampleTime=-1
      settings: Description=|
      | balanceCorrection
      | 
      | WHAT THIS BLOCK DOES
      | Records the input as a MATLAB timeseries for plots and validation. It does not feed a control action back to the robot.
      | 
      | FOLDER CONTEXT
      | RESULTS AND RECORDINGS
      | 
      | Purpose: record signals for plotting and comparison. These blocks do not control the robot.
      | trueState: actual motion; estimatedState: observer output; jointCommand: applied targets.
      | sensorReadout, worldPush and balanceCorrection complete the experiment records.
  estimatedState : ToWorkspace  VariableName=estimatedState  SaveFormat=Timeseries  SampleTime=-1
      settings: Description=|
      | estimatedState
      | 
      | WHAT THIS BLOCK DOES
      | Records the input as a MATLAB timeseries for plots and validation. It does not feed a control action back to the robot.
      | 
      | FOLDER CONTEXT
      | RESULTS AND RECORDINGS
      | 
      | Purpose: record signals for plotting and comparison. These blocks do not control the robot.
      | trueState: actual motion; estimatedState: observer output; jointCommand: applied targets.
      | sensorReadout, worldPush and balanceCorrection complete the experiment records.
  jointCommand : ToWorkspace  VariableName=jointCommand  SaveFormat=Timeseries  SampleTime=-1
      settings: Description=|
      | jointCommand
      | 
      | WHAT THIS BLOCK DOES
      | Records the input as a MATLAB timeseries for plots and validation. It does not feed a control action back to the robot.
      | 
      | FOLDER CONTEXT
      | RESULTS AND RECORDINGS
      | 
      | Purpose: record signals for plotting and comparison. These blocks do not control the robot.
      | trueState: actual motion; estimatedState: observer output; jointCommand: applied targets.
      | sensorReadout, worldPush and balanceCorrection complete the experiment records.
  sensorReadout : ToWorkspace  VariableName=sensorReadout  SaveFormat=Timeseries  SampleTime=-1
      settings: Description=|
      | sensorReadout
      | 
      | WHAT THIS BLOCK DOES
      | Records the input as a MATLAB timeseries for plots and validation. It does not feed a control action back to the robot.
      | 
      | FOLDER CONTEXT
      | RESULTS AND RECORDINGS
      | 
      | Purpose: record signals for plotting and comparison. These blocks do not control the robot.
      | trueState: actual motion; estimatedState: observer output; jointCommand: applied targets.
      | sensorReadout, worldPush and balanceCorrection complete the experiment records.
  trueState : ToWorkspace  VariableName=trueState  SaveFormat=Timeseries  SampleTime=-1
      settings: Description=|
      | trueState
      | 
      | WHAT THIS BLOCK DOES
      | Records the input as a MATLAB timeseries for plots and validation. It does not feed a control action back to the robot.
      | 
      | FOLDER CONTEXT
      | RESULTS AND RECORDINGS
      | 
      | Purpose: record signals for plotting and comparison. These blocks do not control the robot.
      | trueState: actual motion; estimatedState: observer output; jointCommand: applied targets.
      | sensorReadout, worldPush and balanceCorrection complete the experiment records.
  worldPush : ToWorkspace  VariableName=worldPush  SaveFormat=Timeseries  SampleTime=-1
      settings: Description=|
      | worldPush
      | 
      | WHAT THIS BLOCK DOES
      | Records the input as a MATLAB timeseries for plots and validation. It does not feed a control action back to the robot.
      | 
      | FOLDER CONTEXT
      | RESULTS AND RECORDINGS
      | 
      | Purpose: record signals for plotting and comparison. These blocks do not control the robot.
      | trueState: actual motion; estimatedState: observer output; jointCommand: applied targets.
      | sensorReadout, worldPush and balanceCorrection complete the experiment records.
  wires:
  [md8_balanceCorrection] -> balanceCorrection/1
  [md8_estimatedState] -> estimatedState/1
  [md8_jointCommand] -> jointCommand/1
  [md8_sensorReadout] -> sensorReadout/1
  [md8_trueState] -> trueState/1
  [md8_worldPush] -> worldPush/1

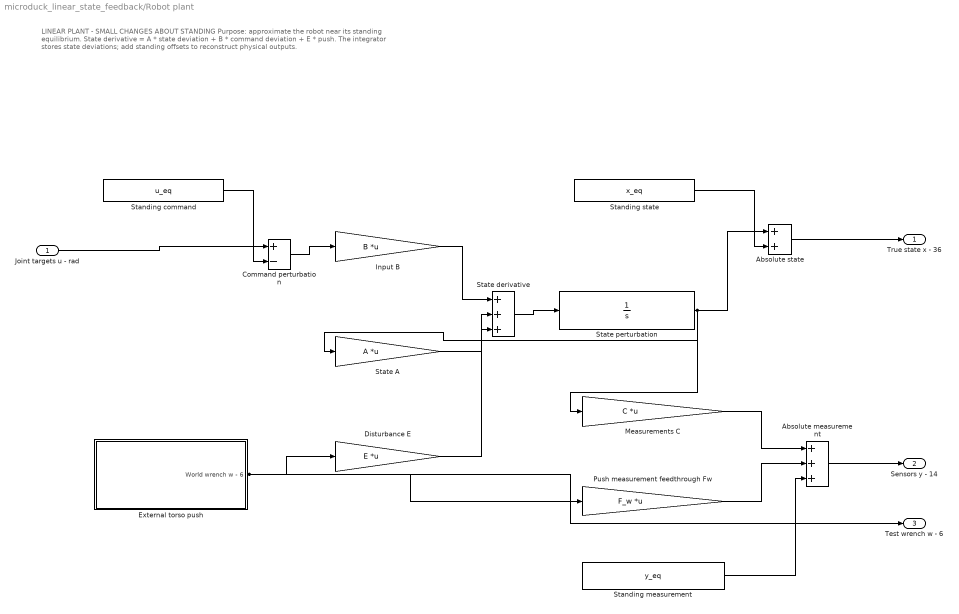
== system microduck_linear_state_feedback/Robot plant ==
  note: LINEAR PLANT - SMALL CHANGES ABOUT STANDING
      |
      | Purpose: approximate the robot near its standing equilibrium.
      | State derivative = A * state deviation + B * command deviation + E * push.
      | The integrator stores state deviations; add standing offsets to reconstruct physical outputs.
  Joint targets u - rad : Inport  Description=|
      | Joint targets u - rad
      | 
      | WHAT THIS BLOCK DOES
      | Receives this named signal from the parent folder. Check the name for its meaning and units.
      | 
      | FOLDER CONTEXT
      | LINEAR PLANT - SMALL CHANGES ABOUT STANDING
      | 
      | Purpose: approximate the robot near its standing equilibrium.
      | State derivative = A * state deviation + B * command deviation + E * push.
      | The integrator stores state deviations; add standing offsets to reconstruct physical outputs.
  Absolute measurement : Sum  Description=|  Inputs=+++
      | Absolute measurement
      | 
      | WHAT THIS BLOCK DOES
      | Combines its inputs using the plus/minus signs shown on the icon. Signs: +++.
      | 
      | FOLDER CONTEXT
      | LINEAR PLANT - SMALL CHANGES ABOUT STANDING
      | 
      | Purpose: approximate the robot near its standing equilibrium.
      | State derivative = A * state deviation + B * command deviation + E * push.
      | The integrator stores state deviations; add standing offsets to reconstruct physical outputs.
  Absolute state : Sum  Description=|
      | Absolute state
      | 
      | WHAT THIS BLOCK DOES
      | Combines its inputs using the plus/minus signs shown on the icon. Signs: ++.
      | 
      | FOLDER CONTEXT
      | LINEAR PLANT - SMALL CHANGES ABOUT STANDING
      | 
      | Purpose: approximate the robot near its standing equilibrium.
      | State derivative = A * state deviation + B * command deviation + E * push.
      | The integrator stores state deviations; add standing offsets to reconstruct physical outputs.
  Command perturbation : Sum  Description=|  Inputs=+-
      | Command perturbation
      | 
      | WHAT THIS BLOCK DOES
      | Combines its inputs using the plus/minus signs shown on the icon. Signs: +-.
      | 
      | FOLDER CONTEXT
      | LINEAR PLANT - SMALL CHANGES ABOUT STANDING
      | 
      | Purpose: approximate the robot near its standing equilibrium.
      | State derivative = A * state deviation + B * command deviation + E * push.
      | The integrator stores state deviations; add standing offsets to reconstruct physical outputs.
  Disturbance E : Gain  Description=|  Gain=E  Multiplication=Matrix(K*u)
      | SHARED PARAMETER: E = r.aux.E
      | Edit sf_parameters.m; per-model edits are refreshed on Run.
      | 
      | WHAT THIS BLOCK DOES
      | Disturbance E
      | 
      | PARAMETER
      | E = r.aux.E
      | 
      | The short symbol is stored in this model workspace. Its numeric value is unchanged from the validated model.
  External torso push : Subsystem  Description=|
      | EXTERNAL TORSO PUSH
      | 
      | Purpose: supply the repeatable disturbance used in this experiment.
      | A Gaussian 0.1 N forward push peaks at 0.2 s, with width 0.02 s.
      | It acts at the torso origin; the observer is not told this disturbance.
      mask help:
      | EXTERNAL TORSO PUSH
      |
      | Purpose: supply the repeatable disturbance used in this experiment.
      | A Gaussian 0.1 N forward push peaks at 0.2 s, with width 0.02 s.
      | It acts at the torso origin; the observer is not told this disturbance.
      settings: OpenFcn=open_system(gcb,'force');
      mask Display: disp('External torso push');
  Input B : Gain  Description=|  Gain=B  Multiplication=Matrix(K*u)
      | SHARED PARAMETER: B = r.lin.B
      | Edit sf_parameters.m; per-model edits are refreshed on Run.
      | 
      | WHAT THIS BLOCK DOES
      | Input B
      | 
      | PARAMETER
      | B = r.lin.B
      | 
      | The short symbol is stored in this model workspace. Its numeric value is unchanged from the validated model.
  Measurements C : Gain  Description=|  Gain=C  Multiplication=Matrix(K*u)
      | SHARED PARAMETER: C = r.lin.C_with_joint_angles
      | Edit sf_parameters.m; per-model edits are refreshed on Run.
      | 
      | WHAT THIS BLOCK DOES
      | Measurements C
      | 
      | PARAMETER
      | C = r.lin.C_with_joint_angles
      | 
      | The short symbol is stored in this model workspace. Its numeric value is unchanged from the validated model.
  Push measurement feedthrough Fw : Gain  Description=|  Gain=F_w  Multiplication=Matrix(K*u)
      | SHARED PARAMETER: F_w = r.aux.Fw
      | Edit sf_parameters.m; per-model edits are refreshed on Run.
      | 
      | WHAT THIS BLOCK DOES
      | Push measurement feedthrough Fw
      | 
      | PARAMETER
      | F_w = r.aux.Fw
      | 
      | The short symbol is stored in this model workspace. Its numeric value is unchanged from the validated model.
  Standing command : Constant  Description=|  Value=u_eq
      | SHARED PARAMETER: u_eq = r.p.ueq
      | Edit sf_parameters.m; per-model edits are refreshed on Run.
      | 
      | WHAT THIS BLOCK DOES
      | Standing command
      | 
      | PARAMETER
      | u_eq = r.p.ueq
      | 
      | The short symbol is stored in this model workspace. Its numeric value is unchanged from the validated model.
  Standing measurement : Constant  Description=|  Value=y_eq
      | SHARED PARAMETER: y_eq = r.observer.y0
      | Edit sf_parameters.m; per-model edits are refreshed on Run.
      | 
      | WHAT THIS BLOCK DOES
      | Standing measurement
      | 
      | PARAMETER
      | y_eq = r.observer.y0
      | 
      | The short symbol is stored in this model workspace. Its numeric value is unchanged from the validated model.
  Standing state : Constant  Description=|  Value=x_eq
      | SHARED PARAMETER: x_eq = r.p.xeq
      | Edit sf_parameters.m; per-model edits are refreshed on Run.
      | 
      | WHAT THIS BLOCK DOES
      | Standing state
      | 
      | PARAMETER
      | x_eq = r.p.xeq
      | 
      | The short symbol is stored in this model workspace. Its numeric value is unchanged from the validated model.
  State A : Gain  Description=|  Gain=A  Multiplication=Matrix(K*u)
      | SHARED PARAMETER: A = r.lin.A
      | Edit sf_parameters.m; per-model edits are refreshed on Run.
      | 
      | WHAT THIS BLOCK DOES
      | State A
      | 
      | PARAMETER
      | A = r.lin.A
      | 
      | The short symbol is stored in this model workspace. Its numeric value is unchanged from the validated model.
  State derivative : Sum  Description=|  Inputs=+++
      | State derivative
      | 
      | WHAT THIS BLOCK DOES
      | Combines its inputs using the plus/minus signs shown on the icon. Signs: +++.
      | 
      | FOLDER CONTEXT
      | LINEAR PLANT - SMALL CHANGES ABOUT STANDING
      | 
      | Purpose: approximate the robot near its standing equilibrium.
      | State derivative = A * state deviation + B * command deviation + E * push.
      | The integrator stores state deviations; add standing offsets to reconstruct physical outputs.
  State perturbation : Integrator  Description=|  InitialCondition=zeros(36,1)
      | State perturbation
      | 
      | WHAT THIS BLOCK DOES
      | Continuous state memory: integrates the input over time. Starts at InitialCondition = zeros(36,1).
      | 
      | FOLDER CONTEXT
      | LINEAR PLANT - SMALL CHANGES ABOUT STANDING
      | 
      | Purpose: approximate the robot near its standing equilibrium.
      | State derivative = A * state deviation + B * command deviation + E * push.
      | The integrator stores state deviations; add standing offsets to reconstruct physical outputs.
  True state x - 36 : Outport  Description=|
      | True state x - 36
      | 
      | WHAT THIS BLOCK DOES
      | Carries this named result out of the folder. The port number defines the interface order.
      | 
      | FOLDER CONTEXT
      | LINEAR PLANT - SMALL CHANGES ABOUT STANDING
      | 
      | Purpose: approximate the robot near its standing equilibrium.
      | State derivative = A * state deviation + B * command deviation + E * push.
      | The integrator stores state deviations; add standing offsets to reconstruct physical outputs.
  Sensors y - 14 : Outport  Description=|  Port=2
      | Sensors y - 14
      | 
      | WHAT THIS BLOCK DOES
      | Carries this named result out of the folder. The port number defines the interface order.
      | 
      | FOLDER CONTEXT
      | LINEAR PLANT - SMALL CHANGES ABOUT STANDING
      | 
      | Purpose: approximate the robot near its standing equilibrium.
      | State derivative = A * state deviation + B * command deviation + E * push.
      | The integrator stores state deviations; add standing offsets to reconstruct physical outputs.
  Test wrench w - 6 : Outport  Description=|  Port=3
      | Test wrench w - 6
      | 
      | WHAT THIS BLOCK DOES
      | Carries this named result out of the folder. The port number defines the interface order.
      | 
      | FOLDER CONTEXT
      | LINEAR PLANT - SMALL CHANGES ABOUT STANDING
      | 
      | Purpose: approximate the robot near its standing equilibrium.
      | State derivative = A * state deviation + B * command deviation + E * push.
      | The integrator stores state deviations; add standing offsets to reconstruct physical outputs.
  wires:
  Measurements C/1 -> Absolute measurement/1
  Push measurement feedthrough Fw/1 -> Absolute measurement/2
  Standing measurement/1 -> Absolute measurement/3
  State perturbation/1 -> Absolute state/1, Measurements C/1, State A/1
  Standing state/1 -> Absolute state/2
  Joint targets u - rad/1 -> Command perturbation/1
  Standing command/1 -> Command perturbation/2
  External torso push/1(World wrench w - 6) -> Disturbance E/1, Push measurement feedthrough Fw/1, Test wrench w - 6/1
  Command perturbation/1 -> Input B/1
  Input B/1 -> State derivative/1
  State A/1 -> State derivative/2
  Disturbance E/1 -> State derivative/3
  State derivative/1 -> State perturbation/1
  Absolute state/1 -> True state x - 36/1
  Absolute measurement/1 -> Sensors y - 14/1

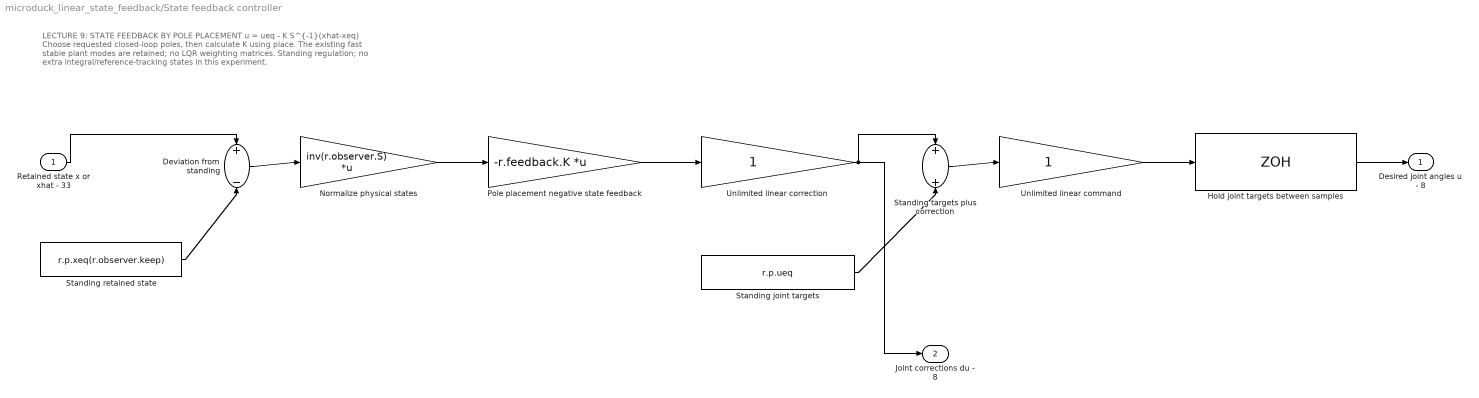
== system microduck_linear_state_feedback/State feedback controller ==
  note: LECTURE 9: STATE FEEDBACK BY POLE PLACEMENT
      | u = ueq - K S^{-1}(xhat-xeq)
      | Choose requested closed-loop poles, then calculate K using place.
      | The existing fast stable plant modes are retained; no LQR weighting matrices.
      | Standing regulation; no extra integral/reference-tracking states in this experiment.
  Retained state x or xhat - 33 : Inport
  Deviation from standing : Sum  Inputs=+-
  Hold joint targets between samples : ZeroOrderHold  Description=Digital controller period Ts. Its input is sampled at the same period as the observer and true-state baseline.  SampleTime=r.observer.sampleTime
  Normalize physical states : Gain  Description=z = S^(-1)*(x-xeq). Scaling makes metres, radians, rates and torques comparable in the LQR cost.  Gain=inv(r.observer.S)  Multiplication=Matrix(K*u)
  Pole placement negative state feedback : Gain  Description=du = -K*z. K is calculated using pole placement in equivalent state coordinates; no LQR cost or weights are used.  Gain=-r.feedback.K  Multiplication=Matrix(K*u)
  Standing joint targets : Constant  Value=r.p.ueq
  Standing retained state : Constant  Value=r.p.xeq(r.observer.keep)
  Standing targets plus correction : Sum
  Unlimited linear command : Gain
  Unlimited linear correction : Gain  Description=The local linear baseline bypasses nonlinear limits, matching the earlier linear plant architecture.
  Desired joint angles u - 8 : Outport
  Joint corrections du - 8 : Outport  Port=2
  wires:
  Retained state x or xhat - 33/1 -> Deviation from standing/1
  Standing retained state/1 -> Deviation from standing/2
  Deviation from standing/1 -> Normalize physical states/1
  Normalize physical states/1 -> Pole placement negative state feedback/1
  Pole placement negative state feedback/1 -> Unlimited linear correction/1
  Unlimited linear correction/1 -> Standing targets plus correction/1, Joint corrections du - 8/1
  Standing joint targets/1 -> Standing targets plus correction/2
  Standing targets plus correction/1 -> Unlimited linear command/1
  Unlimited linear command/1 -> Hold joint targets between samples/1
  Hold joint targets between samples/1 -> Desired joint angles u - 8/1

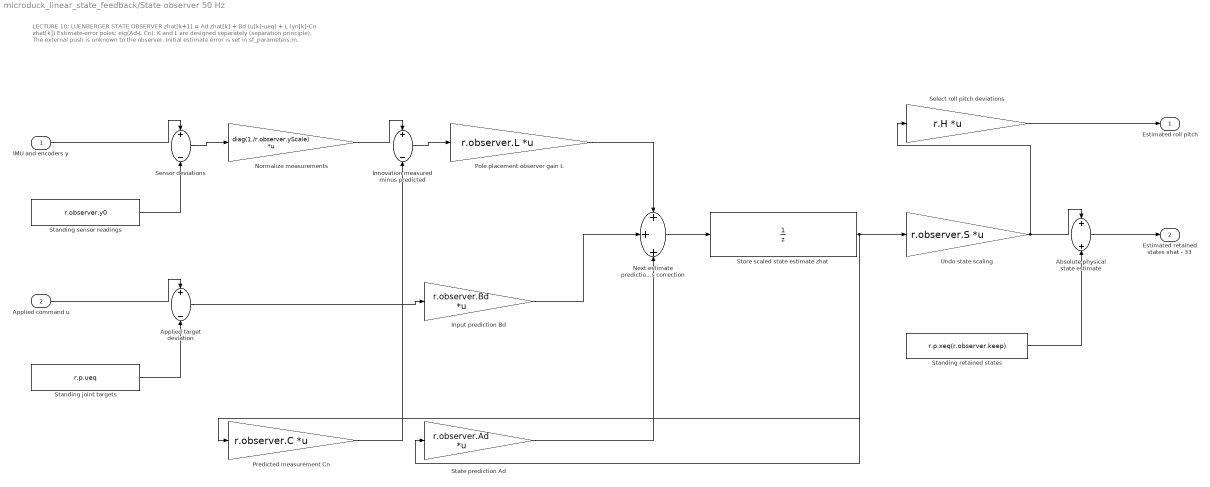
== system microduck_linear_state_feedback/State observer 50 Hz ==
  note: LECTURE 10: LUENBERGER STATE OBSERVER
      | zhat[k+1] = Ad zhat[k] + Bd (u[k]-ueq) + L (yn[k]-Cn zhat[k])
      | Estimate-error poles: eig(Ad-L Cn). K and L are designed separately (separation principle).
      | The external push is unknown to the observer. Initial estimate error is set in sf_parameters.m.
  IMU and encoders y : Inport
  Applied command u : Inport  Port=2
  Absolute physical state estimate : Sum
  Applied target deviation : Sum  Inputs=+-
  Innovation measured minus predicted : Sum  Inputs=+-
  Input prediction Bd : Gain  Description=Bd*(u_applied-ueq). The known input includes outer-controller command limiting.  Gain=r.observer.Bd  Multiplication=Matrix(K*u)
  Next estimate prediction plus correction : Sum  Inputs=+++
  Normalize measurements : Gain  Description=yn = diag(1./yScale)*(y-yeq). Same physical sensors and normalization as the earlier plant.  Gain=diag(1./r.observer.yScale)  Multiplication=Matrix(K*u)
  Pole placement observer gain L : Gain  Description=L*innovation. L is designed by pole placement on the dual system, not by a Kalman filter or covariance weights.  Gain=r.observer.L  Multiplication=Matrix(K*u)
  Predicted measurement Cn : Gain  Gain=r.observer.C  Multiplication=Matrix(K*u)
  Select roll pitch deviations : Gain  Gain=r.H  Multiplication=Matrix(K*u)
  Sensor deviations : Sum  Inputs=+-
  Standing joint targets : Constant  Value=r.p.ueq
  Standing retained states : Constant  Value=r.p.xeq(r.observer.keep)
  Standing sensor readings : Constant  Value=r.observer.y0
  State prediction Ad : Gain  Gain=r.observer.Ad  Multiplication=Matrix(K*u)
  Store scaled state estimate zhat : UnitDelay  Description=Stores zhat[k]. Its input becomes zhat[k+1] at the next sample. This delay makes the observer causal.  InitialCondition=r.observer.S\r.observer.settings.initialEstimateDelta(r.observer.keep)  SampleTime=r.observer.sampleTime
  Undo state scaling : Gain  Gain=r.observer.S  Multiplication=Matrix(K*u)
  Estimated roll pitch : Outport
  Estimated retained states xhat - 33 : Outport  Port=2
  wires:
  IMU and encoders y/1 -> Sensor deviations/1
  Standing sensor readings/1 -> Sensor deviations/2
  Sensor deviations/1 -> Normalize measurements/1
  Normalize measurements/1 -> Innovation measured minus predicted/1
  Predicted measurement Cn/1 -> Innovation measured minus predicted/2
  Innovation measured minus predicted/1 -> Pole placement observer gain L/1
  Applied command u/1 -> Applied target deviation/1
  Standing joint targets/1 -> Applied target deviation/2
  Applied target deviation/1 -> Input prediction Bd/1
  Input prediction Bd/1 -> Next estimate prediction plus correction/2
  Pole placement observer gain L/1 -> Next estimate prediction plus correction/1
  State prediction Ad/1 -> Next estimate prediction plus correction/3
  Next estimate prediction plus correction/1 -> Store scaled state estimate zhat/1
  Store scaled state estimate zhat/1 -> State prediction Ad/1, Predicted measurement Cn/1, Undo state scaling/1
  Undo state scaling/1 -> Absolute physical state estimate/1, Select roll pitch deviations/1
  Standing retained states/1 -> Absolute physical state estimate/2
  Absolute physical state estimate/1 -> Estimated retained states xhat - 33/1
  Select roll pitch deviations/1 -> Estimated roll pitch/1

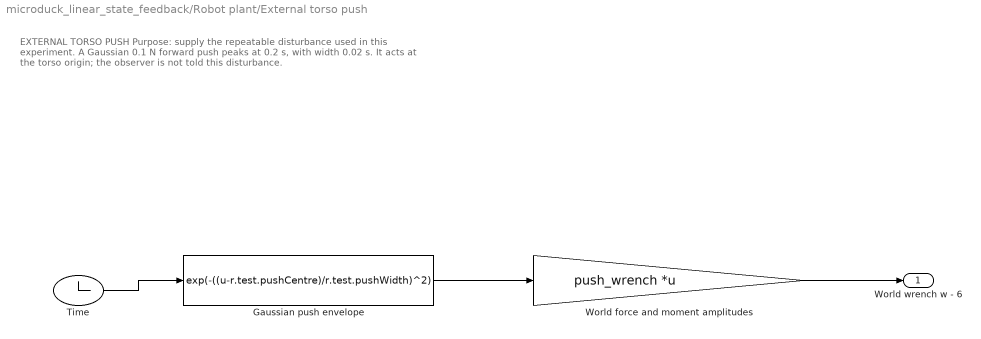
== system microduck_linear_state_feedback/Robot plant/External torso push ==
  note: EXTERNAL TORSO PUSH
      |
      | Purpose: supply the repeatable disturbance used in this experiment.
      | A Gaussian 0.1 N forward push peaks at 0.2 s, with width 0.02 s.
      | It acts at the torso origin; the observer is not told this disturbance.
  Gaussian push envelope : Fcn  Description=|  Expr=exp(-((u-r.test.pushCentre)/r.test.pushWidth)^2)
      | Gaussian push envelope
      | 
      | WHAT THIS BLOCK DOES
      | Performs the mathematical operation named on this block. Open its parameter dialog to inspect the operator and dimensions.
      | 
      | FOLDER CONTEXT
      | EXTERNAL TORSO PUSH
      | 
      | Purpose: supply the repeatable disturbance used in this experiment.
      | A Gaussian 0.1 N forward push peaks at 0.2 s, with width 0.02 s.
      | It acts at the torso origin; the observer is not told this disturbance.
  Time : Clock
      settings: Description=|
      | Time
      | 
      | WHAT THIS BLOCK DOES
      | Performs the mathematical operation named on this block. Open its parameter dialog to inspect the operator and dimensions.
      | 
      | FOLDER CONTEXT
      | EXTERNAL TORSO PUSH
      | 
      | Purpose: supply the repeatable disturbance used in this experiment.
      | A Gaussian 0.1 N forward push peaks at 0.2 s, with width 0.02 s.
      | It acts at the torso origin; the observer is not told this disturbance.
  World force and moment amplitudes : Gain  Description=|  Gain=push_wrench  Multiplication=Matrix(K*u)
      | SHARED PARAMETER: push_wrench = [r.test.pushForce;r.test.pushMoment]
      | Edit sf_parameters.m; per-model edits are refreshed on Run.
      | 
      | WHAT THIS BLOCK DOES
      | World force and moment amplitudes
      | 
      | PARAMETER
      | G13 = [r.test.pushForce;zeros(3,1)]
      | 
      | The short symbol is stored in this model workspace. Its numeric value is unchanged from the validated model.
  World wrench w - 6 : Outport  Description=|
      | World wrench w - 6
      | 
      | WHAT THIS BLOCK DOES
      | Carries this named result out of the folder. The port number defines the interface order.
      | 
      | FOLDER CONTEXT
      | EXTERNAL TORSO PUSH
      | 
      | Purpose: supply the repeatable disturbance used in this experiment.
      | A Gaussian 0.1 N forward push peaks at 0.2 s, with width 0.02 s.
      | It acts at the torso origin; the observer is not told this disturbance.
  wires:
  Time/1 -> Gaussian push envelope/1
  Gaussian push envelope/1 -> World force and moment amplitudes/1
  World force and moment amplitudes/1 -> World wrench w - 6/1
